simulink model "structure_truth"  (R2026b)
settings: Solver=VariableStepAuto
undefined symbols (not defined in the file or in its folder): P
libraries: simulink x4, sharedutil x3
settings Model: Creator=aomar  LastModifiedBy=aomar

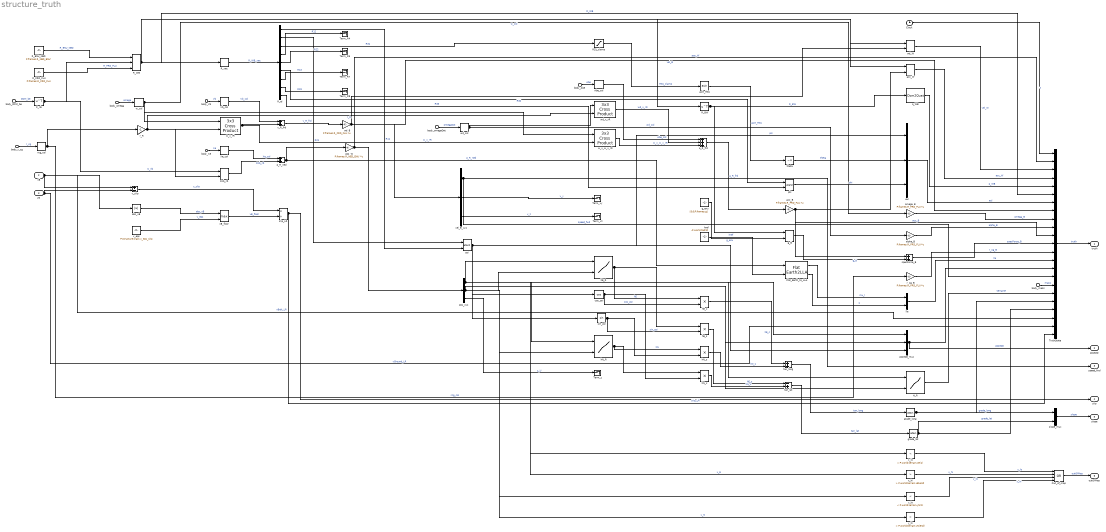
== system structure_truth ==
  body_Xe : Inport  PortName=body  Element=Xe
  body_Vb : Inport  PortName=body  Element=Vb
  body_omega : Inport  PortName=body  Element=omega
  body_omegaDot : Inport  PortName=body  Element=omegaDot
  body_Abe : Inport  PortName=body  Element=Abe
  body_r_cg : Inport  PortName=body  Element=r_cg
  body_DCM_be : Inport  PortName=body  Element=DCM_be
  body_mass : Inport  PortName=body  Element=mass
  vB : Inport  Port=2
  vG : Inport  Port=3
  Abe_col : Reshape  OutputDimensionality=Column vector (2-D)
  C_nb : Math  Operator=transpose
  Clock : Clock
  Cnb_rR : Product  Inputs=**  Multiplication=Matrix(*)
  Flat_Earth_to_LLA : FlatEarth2LLA  LL0=P.world.lla0(1:2)
  H_R : Lookup_n-D  BreakpointsForDimension1=P.world.terrain.xE  BreakpointsForDimension2=P.world.terrain.yN  IndexSearchMethod=Evenly spaced points  Table=P.world.terrain.H  ExtrapMethod=Clip  InternalRulePriority=Speed  RndMeth=Simplest
      settings: InputPortMap=u0,u1
  Out_of_map : Logic  Operator=OR  Inputs=4  AllPortsSameDT=off  OutDataTypeStr=boolean
  R31_clamp : Saturate  UpperLimit=1  LowerLimit=-1
  R_BW : Math  Operator=transpose
  R_ENU_NED : Constant  Value=P.frames.R_NED_ENU'  VectorParams1D=off
  R_FRD_FLU : Constant  Value=P.frames.R_FRD_FLU  VectorParams1D=off
  R_WB : Product  Inputs=***  Multiplication=Matrix(*)
  R_el : Demux  Outputs=9
  R_vec : Reshape
  Term_R{4..5,7..8} (4 alike) : Terminator
  Term_vy : Terminator
  Term_vz : Terminator
  Term_z : Terminator
  TruthState : BusCreator  Inputs=23  OutDataTypeStr=Bus: Bus_TruthState  NonVirtualBus=on
  Vb_col : Reshape  OutputDimensionality=Column vector (2-D)
  Xe_col : Reshape  OutputDimensionality=Column vector (2-D)
  a_R_frd : Sum  Inputs=+++
  abs_vB : Abs  ZeroCross=off  SaturateOnIntegerOverflow=off
  acc_B : Gain  Gain=P.frames.R_FRD_FLU  Multiplication=Matrix(K*u)
  acc_W : Product  Inputs=**  Multiplication=Matrix(*)
  alpha_B : Gain  Gain=P.frames.R_FRD_FLU  Multiplication=Matrix(K*u)
  asin_R31 : Trigonometry  Operator=asin
  cos_psi : Trigonometry  Operator=cos
  eul : Mux  Inputs=3
  g_B : Product  Inputs=**  Multiplication=Matrix(*)
  g_enu : Constant  Value=[0;0;P.frames.g]  VectorParams1D=off
  grade_lat : Trigonometry  Operator=atan
  grade_long : Trigonometry  Operator=atan
  hE_R : Lookup_n-D  BreakpointsForDimension1=P.world.terrain.xE  BreakpointsForDimension2=P.world.terrain.yN  IndexSearchMethod=Evenly spaced points  Table=P.world.terrain.dHdE  ExtrapMethod=Clip  InternalRulePriority=Speed  RndMeth=Simplest
      settings: InputPortMap=u0,u1
  hE_c : Product  Inputs=**
  hE_s : Product  Inputs=**
  hN_R : Lookup_n-D  BreakpointsForDimension1=P.world.terrain.xE  BreakpointsForDimension2=P.world.terrain.yN  IndexSearchMethod=Evenly spaced points  Table=P.world.terrain.dHdN  ExtrapMethod=Clip  InternalRulePriority=Speed  RndMeth=Simplest
      settings: InputPortMap=u0,u1
  hN_c : Product  Inputs=**
  hN_s : Product  Inputs=**
  href : Constant  Value=-P.world.lla0(3)  VectorParams1D=off
  lla : Mux  Inputs=2
  omega_B : Gain  Gain=P.frames.R_FRD_FLU  Multiplication=Matrix(K*u)
  p_R_ned : Sum
  phi : Trigonometry  Operator=atan2
  pos_W : Gain  Gain=P.frames.R_NED_ENU'  Multiplication=Matrix(K*u)
  pos_xyz : Demux  Outputs=3
  pose2D_mux : Mux  Inputs=3
  psi : Trigonometry  Operator=atan2
  q_WB : Dcm2Quat
  r_R : Gain  Gain=-1
  r_cg_B : Gain  Gain=P.frames.R_FRD_FLU  Multiplication=Matrix(K*u)
  rcg_col : Reshape  OutputDimensionality=Column vector (2-D)
  sin_psi : Trigonometry
  slip_LR : Product  Inputs=*/
  slope_mux : Mux  Inputs=2
  specForce_B : Sum
  tan_lat : Sum  Inputs=-+
  tan_long : Sum
  theta : UnaryMinus
  vB_floor : MinMax  Function=max  Inputs=2  ZeroCross=off
  v_R_frd : Sum
  v_eps : Constant  Value=P.structure.track.v_eps_slip  VectorParams1D=off
  v_slip : Sum  Inputs=+-
  vel_B : Gain  Gain=P.frames.R_FRD_FLU  Multiplication=Matrix(K*u)
  vel_B_xyz : Demux  Outputs=3
  vel_W : Product  Inputs=**  Multiplication=Matrix(*)
  w_col : Reshape  OutputDimensionality=Column vector (2-D)
  w_x_rR : sharedutil/3x3 Cross Product  aMode=aMode
      settings: LibrarySourceBlock=aerolibutil/3x3 Cross Product
  w_x_w_x_rR : sharedutil/3x3 Cross Product  aMode=aMode
      settings: LibrarySourceBlock=aerolibutil/3x3 Cross Product
  wd_col : Reshape  OutputDimensionality=Column vector (2-D)
  wd_x_rR : sharedutil/3x3 Cross Product  aMode=aMode
      settings: LibrarySourceBlock=aerolibutil/3x3 Cross Product
  x_hi : simulink/Logic and Bit Operations/Compare To Constant  relop=>  const=P.world.terrain.xE(end)  OutDataTypeStr=boolean
  x_lo : simulink/Logic and Bit Operations/Compare To Constant  relop=<  const=P.world.terrain.xE(1)  OutDataTypeStr=boolean
  y_hi : simulink/Logic and Bit Operations/Compare To Constant  relop=>  const=P.world.terrain.yN(end)  OutDataTypeStr=boolean
  y_lo : simulink/Logic and Bit Operations/Compare To Constant  relop=<  const=P.world.terrain.yN(1)  OutDataTypeStr=boolean
  truth : Outport  OutDataTypeStr=Bus: Bus_TruthState
  pose2D : Outport  Port=2
  speed_fwd : Outport  Port=3
  slip : Outport  Port=4
  slope : Outport  Port=5
  outOfMap : Outport  Port=6
  wires:
  body_DCM_be/1 -> C_nb/1  "DCM_be"
  body_r_cg/1 -> rcg_col/1  "r_cg"
  R_ENU_NED/1 -> R_WB/1  "R_ENU_NED"
  R_FRD_FLU/1 -> R_WB/3  "R_FRD_FLU"
  C_nb/1 -> Cnb_rR/1, R_WB/2  "C_nb"
  rcg_col/1 -> r_cg_B/1, r_R/1  "rcg_col"
  body_omega/1 -> w_col/1  "omega"
  v_slip/1 -> slip_LR/1  "v_slip"
  R_WB/1 -> TruthState/6, R_BW/1, vel_W/1, acc_W/1, R_vec/1  "R_WB"
  abs_vB/1 -> vB_floor/1  "abs_vB"
  v_eps/1 -> vB_floor/2  "v_eps"
  w_col/1 -> omega_B/1, w_x_w_x_rR/1, w_x_rR/1  "w_col"
  r_R/1 -> Cnb_rR/2, wd_x_rR/2, w_x_rR/2  "r_R"
  body_Vb/1 -> Vb_col/1  "Vb"
  body_Xe/1 -> Xe_col/1  "Xe"
  R_vec/1 -> R_el/1  "R_WB_vec"
  Vb_col/1 -> v_R_frd/1  "Vb_col"
  Xe_col/1 -> p_R_ned/1  "Xe_col"
  Cnb_rR/1 -> p_R_ned/2  "Cnb_rR"
  vB_floor/1 -> slip_LR/2  "vB_floor"
  w_x_rR/1 -> w_x_w_x_rR/2, v_R_frd/2  "w_x_rR"
  R_el/1 -> psi/2  "R11"
  R_el/2 -> psi/1  "R21"
  R_el/3 -> R31_clamp/1  "R31"
  R_el/4 -> Term_R4/1  "R12"
  R_el/5 -> Term_R5/1  "R22"
  R_el/6 -> phi/1  "R32"
  R_el/7 -> Term_R7/1  "R13"
  R_el/8 -> Term_R8/1  "R23"
  R_el/9 -> phi/2  "R33"
  v_R_frd/1 -> vel_B/1  "v_R_frd"
  p_R_ned/1 -> Flat_Earth_to_LLA/1, pos_W/1  "p_R_ned"
  slip_LR/1 -> slip/1, TruthState/23  "slip_LR"
  vel_B/1 -> TruthState/8, vel_W/2, vel_B_xyz/1  "vel_B"
  pos_W/1 -> pos_xyz/1, TruthState/2  "pos_W"
  body_omegaDot/1 -> wd_col/1  "omegaDot"
  vel_B_xyz/1 -> speed_fwd/1, TruthState/16  "speed_fwd"
  vel_B_xyz/2 -> Term_vy/1  "v_y"
  vel_B_xyz/3 -> Term_vz/1  "v_z"
  pos_xyz/1 -> x_hi/1, x_lo/1, H_R/1, hN_R/1, pose2D_mux/1, hE_R/1  "x_E"
  pos_xyz/2 -> y_hi/1, y_lo/1, H_R/2, hN_R/2, pose2D_mux/2, hE_R/2  "y_N"
  pos_xyz/3 -> Term_z/1  "z_U"
  wd_col/1 -> alpha_B/1, wd_x_rR/1  "wd_col"
  psi/1 -> eul/1, pose2D_mux/3, sin_psi/1, cos_psi/1  "psi"
  body_Abe/1 -> Abe_col/1  "Abe"
  R31_clamp/1 -> asin_R31/1  "R31_clamp"
  Abe_col/1 -> a_R_frd/1  "Abe_col"
  cos_psi/1 -> hN_c/2, hE_c/2  "cos_psi"
  sin_psi/1 -> hN_s/2, hE_s/2  "sin_psi"
  hE_R/1 -> hE_s/1, hE_c/1  "hE"
  hN_R/1 -> hN_c/1, hN_s/1  "hN"
  wd_x_rR/1 -> a_R_frd/2  "wd_x_rR"
  w_x_w_x_rR/1 -> a_R_frd/3  "w_x_w_x_rR"
  a_R_frd/1 -> acc_B/1  "a_R_frd"
  asin_R31/1 -> theta/1  "asin_R31"
  R_BW/1 -> g_B/1, q_WB/1  "R_BW"
  g_enu/1 -> g_B/2  "g_enu"
  href/1 -> Flat_Earth_to_LLA/2  "href"
  hE_c/1 -> tan_long/1  "hE_c"
  hE_s/1 -> tan_lat/1  "hE_s"
  hN_s/1 -> tan_long/2  "hN_s"
  hN_c/1 -> tan_lat/2  "hN_c"
  tan_long/1 -> grade_long/1  "tan_long"
  tan_lat/1 -> grade_lat/1  "tan_lat"
  theta/1 -> eul/2  "theta"
  phi/1 -> eul/3  "phi"
  acc_B/1 -> acc_W/2, specForce_B/1, TruthState/11  "acc_B"
  g_B/1 -> specForce_B/2  "g_B"
  Flat_Earth_to_LLA/1 -> lla/1  "mu_l"
  Flat_Earth_to_LLA/2 -> lla/2  "h"
  eul/1 -> TruthState/7  "eul"
  lla/1 -> TruthState/14  "lla"
  pose2D_mux/1 -> TruthState/15, pose2D/1  "pose2D"
  Clock/1 -> TruthState/1  "t"
  specForce_B/1 -> TruthState/12  "specForce_B"
  vel_W/1 -> TruthState/3  "vel_W"
  acc_W/1 -> TruthState/4  "acc_W"
  omega_B/1 -> TruthState/9  "omega_B"
  alpha_B/1 -> TruthState/10  "alpha_B"
  r_cg_B/1 -> TruthState/13  "r_cg_B"
  grade_long/1 -> TruthState/19, slope_mux/1  "grade_long"
  x_lo/1 -> Out_of_map/1  "x_lo"
  x_hi/1 -> Out_of_map/2  "x_hi"
  y_lo/1 -> Out_of_map/3  "y_lo"
  y_hi/1 -> Out_of_map/4  "y_hi"
  grade_lat/1 -> TruthState/20, slope_mux/2  "grade_lat"
  q_WB/1 -> TruthState/5  "q_WB"
  H_R/1 -> TruthState/18  "terrainH"
  body_mass/1 -> TruthState/17  "mass"
  TruthState/1 -> truth/1  "truth"
  slope_mux/1 -> slope/1  "slope"
  Out_of_map/1 -> outOfMap/1  "outOfMap"
  vB/1 -> TruthState/21, abs_vB/1, v_slip/1  "vBelt_LR"
  vG/1 -> TruthState/22, v_slip/2  "vGround_LR"
